simulink model "labaZB"  (R2022a)
settings: Solver=VariableStepAuto  StartTime=0.0  StopTime=10  RelTol=1e-3
settings Model: Creator=User  LastModifiedBy=salgi

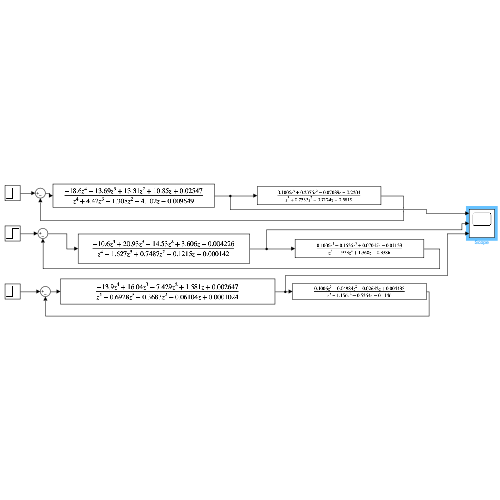
[thumbnail: Simulink's stored preview of the top-level diagram]
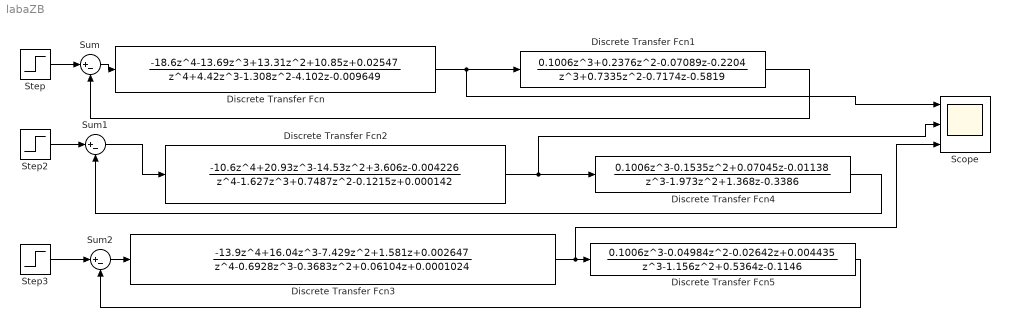
== system labaZB ==
  Discrete Transfer Fcn : DiscreteTransferFcn  Numerator=[-18.6 -13.69 13.31 10.85 0.02547]  Denominator=[1 4.42 -1.308 -4.102 -0.009649]
  Discrete Transfer Fcn1 : DiscreteTransferFcn  Numerator=[0.1006 0.2376 -0.07089 -0.2204]  Denominator=[1 0.7335 -0.7174 -0.5819]
  Discrete Transfer Fcn2 : DiscreteTransferFcn  Numerator=[-10.6 20.93 -14.53 3.606 -0.004226]  Denominator=[1 -1.627 0.7487 -0.1215 0.000142]
  Discrete Transfer Fcn3 : DiscreteTransferFcn  Numerator=[-13.9 16.04 -7.429 1.581 0.002647]  Denominator=[1 -0.6928 -0.3683 0.06104 0.0001024]
  Discrete Transfer Fcn4 : DiscreteTransferFcn  Numerator=[0.1006 -0.1535 0.07045 -0.01138]  Denominator=[1 -1.973 1.368 -0.3386]
  Discrete Transfer Fcn5 : DiscreteTransferFcn  Numerator=[0.1006 -0.04984 -0.02642 0.004435]  Denominator=[1 -1.156 0.5364 -0.1146]
  Scope : Scope  NumInputPorts=3
  Step : Step  SampleTime=1
  Step2 : Step  SampleTime=2
  Step3 : Step  SampleTime=4
  Sum : Sum  Inputs=|+-
  Sum1 : Sum  Inputs=|+-
  Sum2 : Sum  Inputs=|+-
  wires:
  Step/1 -> Sum/1
  Sum/1 -> Discrete Transfer Fcn/1
  Discrete Transfer Fcn/1 -> Discrete Transfer Fcn1/1, Scope/1
  Discrete Transfer Fcn1/1 -> Sum/2
  Discrete Transfer Fcn2/1 -> Scope/2, Discrete Transfer Fcn4/1
  Sum1/1 -> Discrete Transfer Fcn2/1
  Discrete Transfer Fcn3/1 -> Scope/3, Discrete Transfer Fcn5/1
  Sum2/1 -> Discrete Transfer Fcn3/1
  Discrete Transfer Fcn4/1 -> Sum1/2
  Discrete Transfer Fcn5/1 -> Sum2/2
  Step2/1 -> Sum1/1
  Step3/1 -> Sum2/1
